simulink model "Factory_Physics_Model_final_harness"  (R2024b)
settings: Solver=ode4  StartTime=0  StopTime=45  FixedStep=0.0005  RelTol=1e-3
libraries: SignalEditorBlockLib x1
settings Model: Creator=shash  LastModifiedBy=shash
settings ModelReferenceCC: ModelReferenceNumInstancesAllowed=Single

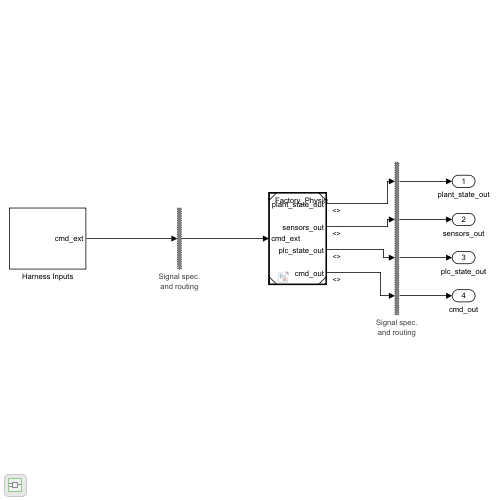
[thumbnail: Simulink's stored preview of the top-level diagram]
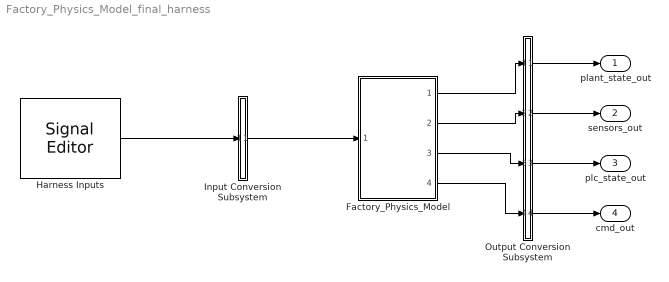
== system Factory_Physics_Model_final_harness ==
  Factory_Physics_Model : ModelReference  ModelNameDialog=Factory_Physics_Model  SimulationMode=Normal  ModelReferenceVersion=1.1
  Harness Inputs : SignalEditorBlockLib/Signal Editor  FileName=C:\Users\shash\Desktop\WILP Work\Digital Twin\Factory_Simulation\Factory_Simulation\slprj\mbd_agent\test\Factory_Physics_Model\Factory_Physics_Model_final_harness_HarnessInputs.mat  ActiveScenario=InputScenario  ActiveSignal=cmd_ext  IsBus=off  OutputBusObjectStr=Bus: BusObject  SampleTime=0  Interpolate=off  ZeroCross=off  OutputAfterFinalValue=Setting to zero  Unit=inherit  PreserveSignalName=on  ApplySigPropsToAllScenarios=on  ApplySigPropsToAllSignals=off
  Input Conversion Subsystem : Subsystem  Tag=__SLT_ICS__  Description=|
      | Signal spec.
      | and routing
      settings: AttributesFormatString=%<Description>
  Output Conversion Subsystem : Subsystem  Tag=__SLT_OCS__  Description=|
      | Signal spec.
      | and routing
      settings: AttributesFormatString=%<Description>
  plant_state_out : Outport
  sensors_out : Outport  Port=2
  plc_state_out : Outport  Port=3
  cmd_out : Outport  Port=4
  wires:
  Harness Inputs/1 -> Input Conversion Subsystem/1(Inport_1)
  Output Conversion Subsystem/1(Outport_1) -> plant_state_out/1
  Output Conversion Subsystem/2(Outport_2) -> sensors_out/1
  Output Conversion Subsystem/3(Outport_3) -> plc_state_out/1
  Output Conversion Subsystem/4(Outport_4) -> cmd_out/1
  Input Conversion Subsystem/1(Outport_1) -> Factory_Physics_Model/1
  Factory_Physics_Model/1 -> Output Conversion Subsystem/1(Inport_1)
  Factory_Physics_Model/2 -> Output Conversion Subsystem/2(Inport_2)
  Factory_Physics_Model/3 -> Output Conversion Subsystem/3(Inport_3)
  Factory_Physics_Model/4 -> Output Conversion Subsystem/4(Inport_4)

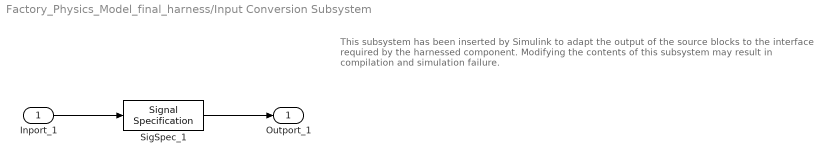
== system Factory_Physics_Model_final_harness/Input Conversion Subsystem ==
  note: This subsystem has been inserted by Simulink to adapt the output of the source blocks to the interface required by the harnessed component.
      |  Modifying the contents of this subsystem may result in compilation and simulation failure.
  Inport_1 : Inport
  SigSpec_1 : SignalSpecification  OutDataTypeStr=double  Dimensions=[14]  SampleTime=[0, 0]
  Outport_1 : Outport
  wires:
  SigSpec_1/1 -> Outport_1/1
  Inport_1/1 -> SigSpec_1/1

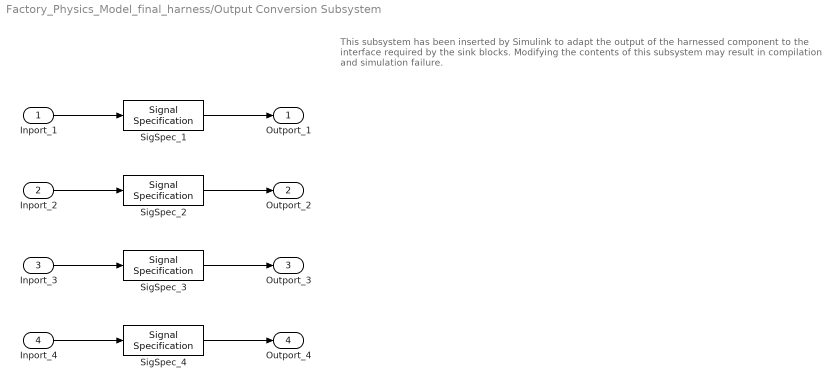
== system Factory_Physics_Model_final_harness/Output Conversion Subsystem ==
  note: This subsystem has been inserted by Simulink to adapt the output of the harnessed component to the interface required by the sink blocks.
      |  Modifying the contents of this subsystem may result in compilation and simulation failure.
  Inport_1 : Inport
  Inport_2 : Inport  Port=2
  Inport_3 : Inport  Port=3
  Inport_4 : Inport  Port=4
  SigSpec_1 : SignalSpecification  OutDataTypeStr=double  Dimensions=[51]
  SigSpec_2 : SignalSpecification  OutDataTypeStr=double  Dimensions=[28]
  SigSpec_3 : SignalSpecification  OutDataTypeStr=double  Dimensions=[1]  SampleTime=0.01
  SigSpec_4 : SignalSpecification  OutDataTypeStr=double  Dimensions=[14]
  Outport_1 : Outport
  Outport_2 : Outport  Port=2
  Outport_3 : Outport  Port=3
  Outport_4 : Outport  Port=4
  wires:
  Inport_1/1 -> SigSpec_1/1
  SigSpec_1/1 -> Outport_1/1
  Inport_2/1 -> SigSpec_2/1
  SigSpec_2/1 -> Outport_2/1
  Inport_3/1 -> SigSpec_3/1
  SigSpec_3/1 -> Outport_3/1
  Inport_4/1 -> SigSpec_4/1
  SigSpec_4/1 -> Outport_4/1
